simulink model "HDLCrestFactorReduction"  (R2026a)
settings: Solver=FixedStepDiscrete  StopTime=stopTime
values from neighbouring files (symbols this model uses):
  ofdmSampleRate = scs*1e3*Nfft    (= 1920000)    [CrestFactorReductionHDL.m]
  threshold = 0.7    [CrestFactorReductionHDL.m]
libraries: dspsrcs4 x2, simulink x1
settings Model: DataTypeOverride=Off  Creator=The MathWorks, Inc.  LastModifiedBy=taokhe
settings OptimizationCC: ConditionallyExecuteInputs=off  InheritOutputTypeSmallerThanSingle=on
settings DebuggingCC: ArtificialAlgebraicLoopMsg=error  SingleTaskRateTransMsg=error
settings HardwareCC: ProdHWDeviceType=ASIC/FPGA->ASIC/FPGA  TargetBitPerLong=64.0  TargetBitPerPointer=64.0  TargetBitPerSizeT=64.0  TargetBitPerPtrDiffT=64.0  TargetLongLongMode=on  TargetIntDivRoundTo=Zero  TargetEndianess=LittleEndian  TargetWordSize=64.0  TargetHWDeviceType=Custom Processor->MATLAB Host Computer  ProdEqTarget=off

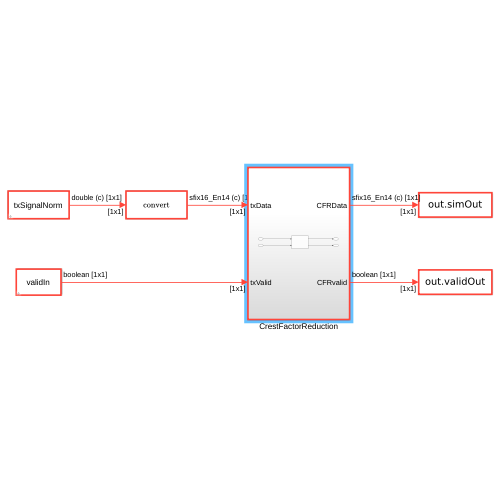
[thumbnail: Simulink's stored preview of the top-level diagram]
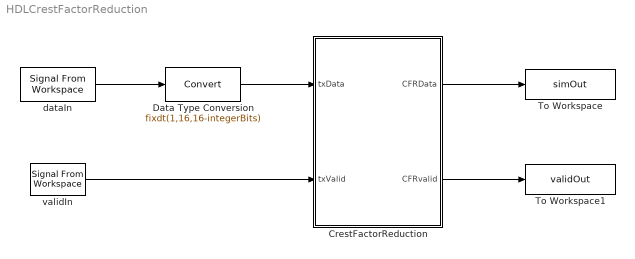
== system HDLCrestFactorReduction ==
  CrestFactorReduction : Subsystem
  Data Type Conversion : DataTypeConversion  OutDataTypeStr=fixdt(1,16,16-integerBits)  SaturateOnIntegerOverflow=off  RndMeth=Floor
  To Workspace : ToWorkspace  VariableName=simOut  SampleTime=-1
      settings: Save2DSignal=2-D array (concatenate along first dimension)
  To Workspace1 : ToWorkspace  VariableName=validOut  SampleTime=-1
      settings: Save2DSignal=2-D array (concatenate along first dimension)
  dataIn : dspsrcs4/Signal From Workspace  X=txSignalNorm  Ts=1/ofdmSampleRate  nsamps=1  OutputAfterFinalValue=Setting to zero  ignoreOrWarnInputAndFrameLengths=off  OutputFrames=off
  validIn : dspsrcs4/Signal From Workspace  X=validIn  Ts=1/ofdmSampleRate  nsamps=1  OutputAfterFinalValue=Setting to zero  ignoreOrWarnInputAndFrameLengths=off  OutputFrames=off
  wires:
  dataIn/1 -> Data Type Conversion/1
  CrestFactorReduction/1(CFRData) -> To Workspace/1
  CrestFactorReduction/2(CFRvalid) -> To Workspace1/1
  Data Type Conversion/1 -> CrestFactorReduction/1(txData)
  validIn/1 -> CrestFactorReduction/2(txValid)

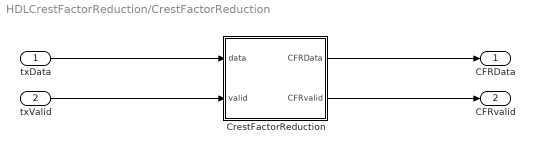
== system HDLCrestFactorReduction/CrestFactorReduction ==
  txData : Inport
  txValid : Inport  Port=2
  CrestFactorReduction : Subsystem  mask{Threshold=threshold}
  CFRData : Outport
  CFRvalid : Outport  Port=2
  wires:
  txData/1 -> CrestFactorReduction/1(data)
  txValid/1 -> CrestFactorReduction/2(valid)
  CrestFactorReduction/1(CFRData) -> CFRData/1
  CrestFactorReduction/2(CFRvalid) -> CFRvalid/1

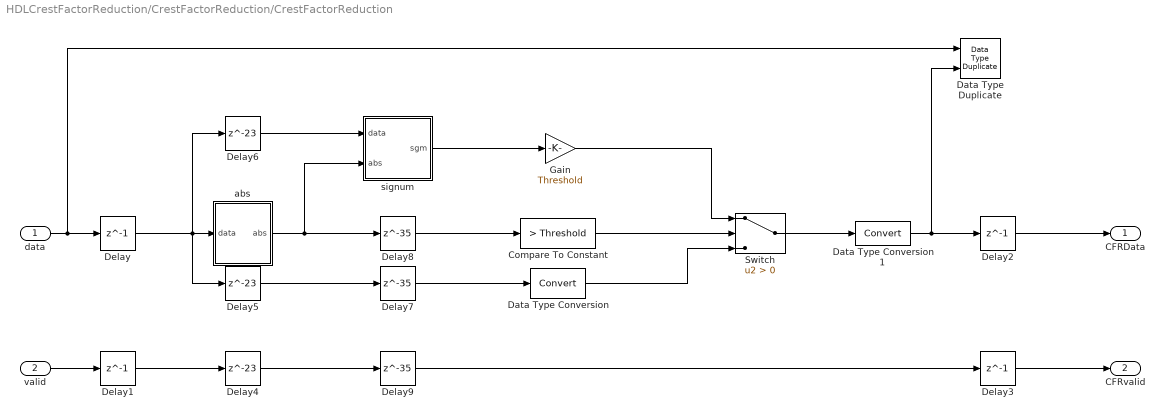
== system HDLCrestFactorReduction/CrestFactorReduction/CrestFactorReduction ==
  data : Inport
  valid : Inport  Port=2
  Compare To Constant : simulink/Logic and Bit Operations/Compare To Constant  relop=>  const=Threshold  OutDataTypeStr=boolean
  Data Type Duplicate : DataTypeDuplicate
  Data Type Conversion : DataTypeConversion  SaturateOnIntegerOverflow=off  RndMeth=Floor
  Data Type Conversion1 : DataTypeConversion  SaturateOnIntegerOverflow=off  RndMeth=Floor
  Delay{,1..3} (4 alike) : Delay  DelayLength=1
  Delay4 : Delay  DelayLength=23
  Delay5 : Delay  DelayLength=23
  Delay6 : Delay  DelayLength=23
  Delay7 : Delay  DelayLength=35
  Delay8 : Delay  DelayLength=35
  Delay9 : Delay  DelayLength=35
  Gain : Gain  Gain=Threshold
  Switch : Switch  Criteria=u2 > Threshold  SaturateOnIntegerOverflow=off  InputSameDT=off
  abs : Subsystem
  signum : Subsystem
  CFRData : Outport
  CFRvalid : Outport  Port=2
  wires:
  data/1 -> Data Type Duplicate/1, Delay/1
  Compare To Constant/1 -> Switch/2
  Switch/1 -> Data Type Conversion1/1
  valid/1 -> Delay1/1
  abs/1(abs) -> signum/2(abs), Delay8/1
  Delay/1 -> Delay6/1, abs/1(data), Delay5/1
  Delay1/1 -> Delay4/1
  Delay2/1 -> CFRData/1
  Delay3/1 -> CFRvalid/1
  Data Type Conversion/1 -> Switch/3
  signum/1(sgm) -> Gain/1
  Gain/1 -> Switch/1
  Delay4/1 -> Delay9/1
  Delay5/1 -> Delay7/1
  Delay6/1 -> signum/1(data)
  Delay7/1 -> Data Type Conversion/1
  Delay8/1 -> Compare To Constant/1
  Delay9/1 -> Delay3/1
  Data Type Conversion1/1 -> Data Type Duplicate/2, Delay2/1

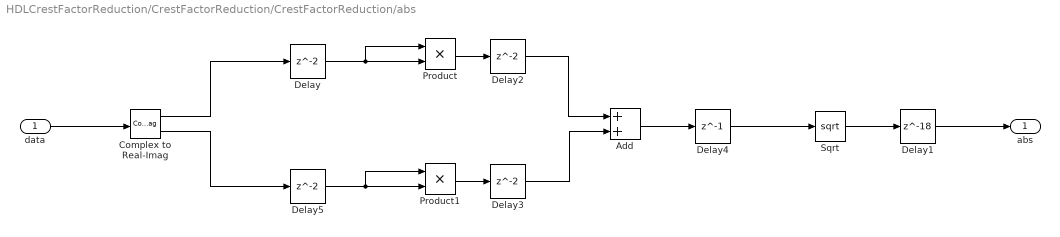
== system HDLCrestFactorReduction/CrestFactorReduction/CrestFactorReduction/abs ==
  data : Inport
  Add : Sum
  Complex to Real-Imag : ComplexToRealImag
  Delay{,2..3,5} (4 alike) : Delay
  Delay1 : Delay  DelayLength=18
  Delay4 : Delay  DelayLength=1
  Product : Product
  Product1 : Product
  Sqrt : Sqrt  OutDataTypeStr=Inherit: Inherit via internal rule
  abs : Outport
  wires:
  Complex to Real-Imag/1 -> Delay/1
  Complex to Real-Imag/2 -> Delay5/1
  Product/1 -> Delay2/1
  Product1/1 -> Delay3/1
  Add/1 -> Delay4/1
  Sqrt/1 -> Delay1/1
  data/1 -> Complex to Real-Imag/1
  Delay1/1 -> abs/1
  Delay2/1 -> Add/1
  Delay3/1 -> Add/2
  Delay4/1 -> Sqrt/1
  Delay/1 -> Product/1, Product/2
  Delay5/1 -> Product1/1, Product1/2

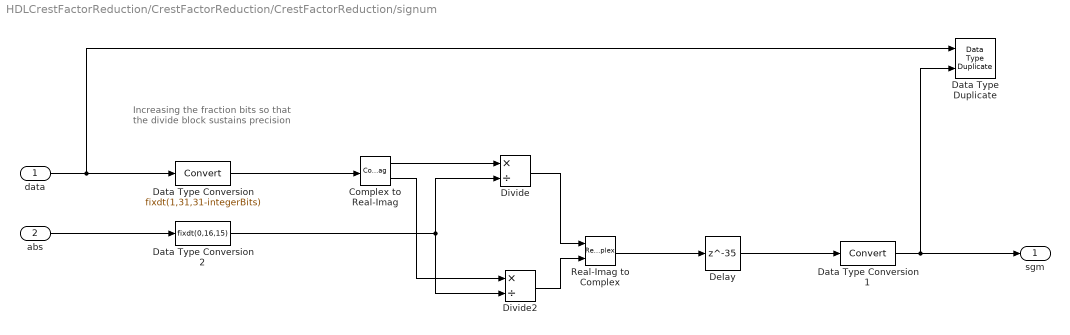
== system HDLCrestFactorReduction/CrestFactorReduction/CrestFactorReduction/signum ==
  note: Increasing the fraction bits so that
      | the divide block sustains precision
  data : Inport
  abs : Inport  Port=2
  Complex to Real-Imag : ComplexToRealImag
  Data Type Duplicate : DataTypeDuplicate
  Data Type Conversion : DataTypeConversion  OutDataTypeStr=fixdt(1,31,31-integerBits)  SaturateOnIntegerOverflow=off  RndMeth=Floor
  Data Type Conversion1 : DataTypeConversion  SaturateOnIntegerOverflow=off  RndMeth=Floor
  Data Type Conversion2 : DataTypeConversion  OutDataTypeStr=fixdt(0,16,15)  SaturateOnIntegerOverflow=off  RndMeth=Floor
  Delay : Delay  DelayLength=35
  Divide : Product  Inputs=*/  RndMeth=Zero  SaturateOnIntegerOverflow=on
  Divide2 : Product  Inputs=*/  RndMeth=Zero  SaturateOnIntegerOverflow=on
  Real-Imag to Complex : RealImagToComplex
  sgm : Outport
  wires:
  data/1 -> Data Type Duplicate/1, Data Type Conversion/1
  Data Type Conversion/1 -> Complex to Real-Imag/1
  Complex to Real-Imag/1 -> Divide/1
  Complex to Real-Imag/2 -> Divide2/1
  Divide/1 -> Real-Imag to Complex/1
  Divide2/1 -> Real-Imag to Complex/2
  Real-Imag to Complex/1 -> Delay/1
  Delay/1 -> Data Type Conversion1/1
  Data Type Conversion1/1 -> Data Type Duplicate/2, sgm/1
  abs/1 -> Data Type Conversion2/1
  Data Type Conversion2/1 -> Divide2/2, Divide/2
